simulink model "pruebaLM386"  (R2023b)
settings: Solver=VariableStepAuto  StartTime=0.0  StopTime=10.0  RelTol=1e-3
libraries: fl_lib x28, ee_lib x11, nesl_utility x3, slctrl_linear x1
settings Model: Creator=Elias  LastModifiedBy=Elias

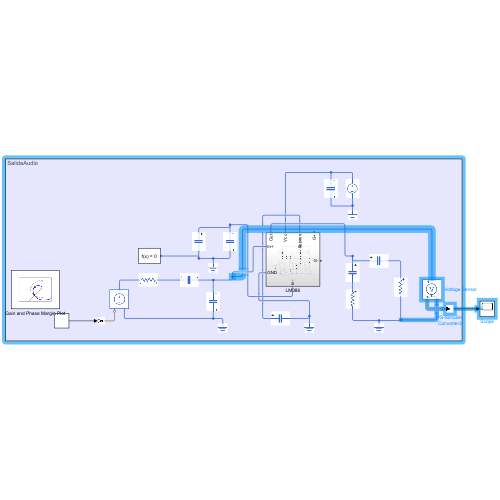
[thumbnail: Simulink's stored preview of the top-level diagram]
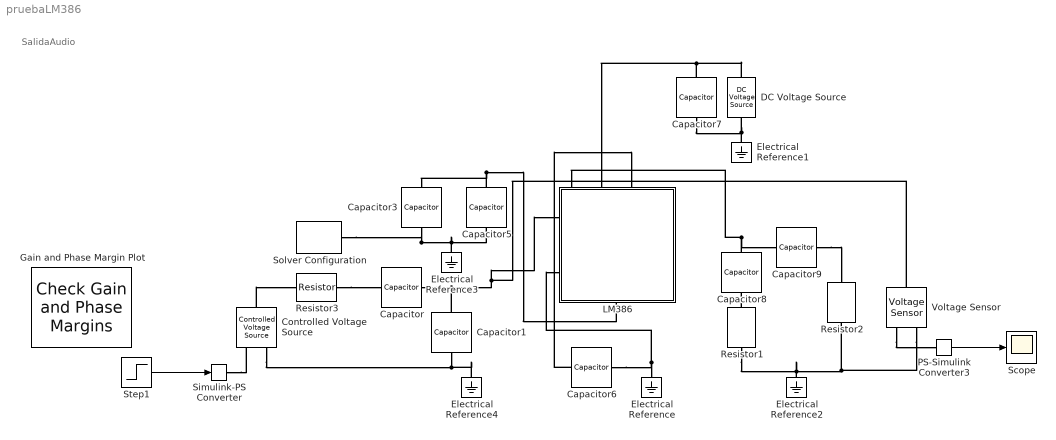
== system pruebaLM386 ==
  note: SalidaAudio
  Capacitor : fl_lib/Electrical/Electrical Elements/Capacitor  c=470e-9 F  r=0 Ohm  g=0 1/Ohm  i_specify=off  i_priority=None  i=0 A  i_nominal_specify=off  i_nominal_unit=A  i_nominal_value=1  v_specify=off  v_priority=None  v=0 V  v_nominal_specify=off  v_nominal_unit=V  v_nominal_value=1  vc_specify=off  vc_priority=High  vc=0 V  vc_nominal_specify=off  vc_nominal_unit=V  vc_nominal_value=1
  Capacitor1 : fl_lib/Electrical/Electrical Elements/Capacitor  c=1e-9 F  r=0 Ohm  g=0 1/Ohm  i_specify=off  i_priority=None  i=0 A  i_nominal_specify=off  i_nominal_unit=A  i_nominal_value=1  v_specify=off  v_priority=None  v=0 V  v_nominal_specify=off  v_nominal_unit=V  v_nominal_value=1  vc_specify=off  vc_priority=High  vc=0 V  vc_nominal_specify=off  vc_nominal_unit=V  vc_nominal_value=1
  Capacitor3 : fl_lib/Electrical/Electrical Elements/Capacitor  c=470e-9 F  r=0 Ohm  g=0 1/Ohm  i_specify=off  i_priority=None  i=0 A  i_nominal_specify=off  i_nominal_unit=A  i_nominal_value=1  v_specify=off  v_priority=None  v=0 V  v_nominal_specify=off  v_nominal_unit=V  v_nominal_value=1  vc_specify=off  vc_priority=High  vc=0 V  vc_nominal_specify=off  vc_nominal_unit=V  vc_nominal_value=1
  Capacitor5 : fl_lib/Electrical/Electrical Elements/Capacitor  c=1e-9 F  r=0 Ohm  g=0 1/Ohm  i_specify=off  i_priority=None  i=0 A  i_nominal_specify=off  i_nominal_unit=A  i_nominal_value=1  v_specify=off  v_priority=None  v=0 V  v_nominal_specify=off  v_nominal_unit=V  v_nominal_value=1  vc_specify=off  vc_priority=High  vc=0 V  vc_nominal_specify=off  vc_nominal_unit=V  vc_nominal_value=1
  Capacitor6 : fl_lib/Electrical/Electrical Elements/Capacitor  c=100e-6 F  r=0 Ohm  g=0 1/Ohm  i_specify=off  i_priority=None  i=0 A  i_nominal_specify=off  i_nominal_unit=A  i_nominal_value=1  v_specify=off  v_priority=None  v=0 V  v_nominal_specify=off  v_nominal_unit=V  v_nominal_value=1  vc_specify=off  vc_priority=High  vc=0 V  vc_nominal_specify=off  vc_nominal_unit=V  vc_nominal_value=1
  Capacitor7 : fl_lib/Electrical/Electrical Elements/Capacitor  c=100e-6 F  r=0 Ohm  g=0 1/Ohm  i_specify=off  i_priority=None  i=0 A  i_nominal_specify=off  i_nominal_unit=A  i_nominal_value=1  v_specify=off  v_priority=None  v=0 V  v_nominal_specify=off  v_nominal_unit=V  v_nominal_value=1  vc_specify=off  vc_priority=High  vc=0 V  vc_nominal_specify=off  vc_nominal_unit=V  vc_nominal_value=1
  Capacitor8 : fl_lib/Electrical/Electrical Elements/Capacitor  c=47e-6 F  r=0 Ohm  g=0 1/Ohm  i_specify=off  i_priority=None  i=0 A  i_nominal_specify=off  i_nominal_unit=A  i_nominal_value=1  v_specify=off  v_priority=None  v=0 V  v_nominal_specify=off  v_nominal_unit=V  v_nominal_value=1  vc_specify=off  vc_priority=High  vc=0 V  vc_nominal_specify=off  vc_nominal_unit=V  vc_nominal_value=1
  Capacitor9 : fl_lib/Electrical/Electrical Elements/Capacitor  c=3.3e-3 F  r=0 Ohm  g=0 1/Ohm  i_specify=off  i_priority=None  i=0 A  i_nominal_specify=off  i_nominal_unit=A  i_nominal_value=1  v_specify=off  v_priority=None  v=0 V  v_nominal_specify=off  v_nominal_unit=V  v_nominal_value=1  vc_specify=off  vc_priority=High  vc=0 V  vc_nominal_specify=off  vc_nominal_unit=V  vc_nominal_value=1
  Controlled Voltage Source : fl_lib/Electrical/Electrical Sources/Controlled Voltage Source
  DC Voltage Source : fl_lib/Electrical/Electrical Sources/DC Voltage Source  v0=5 V
  Electrical Reference{,1..4} (5 alike) : fl_lib/Electrical/Electrical Elements/Electrical Reference
  Gain and Phase Margin Plot : slctrl_linear/Check Gain and Phase Margins  InstantiateOnLoad=on  SaveOperatingPoints=off  LinearizationIOs={'/Step1', 1, 'in', 'off', '';'/PS-Simulink Converter3', 1, 'out', 'on', ''}  LinearizeAt=SnapshotTimes  SnapshotTimes=[0]  TriggerType=rising  SampleTime=auto  RateConversionMethod=zoh  PreWarpFreq=10  UseExactDelayModel=off  UseFullBlockNameLabels=off  UseBusSignalLabels=off  enabled=on  stopWhenAssertionFail=off  export=off  ViewDlgPos=[1 49 1536 740.8]  LaunchViewOnOpen=off  OpenViewOnLoad=on  FrequencyUnits=rad/s  MagnitudeUnits=dB  PhaseUnits=deg  TimeUnits=seconds  EnableMargins=off  GainMargin=[]  PhaseMargin=[]  PlotType=bode  FeedbackSign=-1
      settings: LibrarySourceBlock=slctrlblks/Linear Analysis Plots/Gain and Phase Margin Plot  SaveToWorkspace=off  SaveName=sys
  LM386 : Subsystem
      settings: PortSchema="{\"entries\":[{\"content\":{\"sides\":[{\"content\":{\"connectorIds\":[\"LConn1\",\"LConn2\"]},\"type\":\"ConnectorPlacement.EquallySpacedRectSide\",\"uuid\":\"2337400e-b5e6-493f-9361-1980809f2d02\"},{\"content\":{\"connectorIds\":[\"RConn1\"],\"side\":\"RIGHT\"},\"type\":\"ConnectorPlacement.EquallySpacedRectSide\",\"uuid\":\"8454aa5c-1d69-40e4-a810-e77be7f85d5b\"},{\"content\":{\"connectorIds\":[\"LConn3\",\"LConn4\",\"LConn5\",\"LConn6\"],\"side\":\"TOP\"},\"type\":\"ConnectorPlacement.EquallySpacedRectSide\",\"uuid\":\"a2e8fa12-598a-43b9-9543-b1b71967ef13\"},{\"content\":{\"connectorIds\":[\"RConn2\"],\"side\":\"BOTTOM\"},\"type\":\"ConnectorPlacement.EquallySpacedRectSide\",\"uuid\":\"694fd00f-bc4d-4e22-a44d-beff6c6d18ee\"}]},\"type\":\"ConnectorPlacement.EquallySpacedConnector\",\"uuid\":\"d8918919-7b49-430f-8ddf-b4266ff1b5a4\"}],\"packageUris\":[\"http://schema.mathworks.com/mf0/Connector/R2020b\"],\"version\":\"1.0\"}"
  PS-Simulink Converter3 : nesl_utility/PS-Simulink Converter  PhysicalDomain=network_engine_domain  SubClassName=ps_output  LeftPortType=input  RightPortType=output  PseudoPeriodic=off  Frequencies=[]  VectorFormat=inherit  Unit=inherit  AffineConversion=off
  Resistor1 : fl_lib/Electrical/Electrical Elements/Resistor  R=10 Ohm  i_specify=off  i_priority=None  i=0 A  i_nominal_specify=off  i_nominal_unit=A  i_nominal_value=1  v_specify=off  v_priority=None  v=0 V  v_nominal_specify=off  v_nominal_unit=V  v_nominal_value=1
  Resistor2 : fl_lib/Electrical/Electrical Elements/Resistor  R=8 Ohm  i_specify=off  i_priority=None  i=0 A  i_nominal_specify=off  i_nominal_unit=A  i_nominal_value=1  v_specify=off  v_priority=None  v=0 V  v_nominal_specify=off  v_nominal_unit=V  v_nominal_value=1
  Resistor3 : fl_lib/Electrical/Electrical Elements/Resistor  R=47 Ohm  i_specify=off  i_priority=None  i=0 A  i_nominal_specify=off  i_nominal_unit=A  i_nominal_value=1  v_specify=off  v_priority=None  v=0 V  v_nominal_specify=off  v_nominal_unit=V  v_nominal_value=1
  Scope : Scope
  Simulink-PS Converter : nesl_utility/Simulink-PS Converter  PhysicalDomain=network_engine_domain  SubClassName=ps_input  LeftPortType=input  RightPortType=output  PseudoPeriodic=off  Frequencies=[]  NoiseDistribution=none  NoiseParameters=[]  Unit=1  AffineConversion=on  FilteringAndDerivatives=filter  SimscapeFilterOrder=1  InputFilterTimeConstant=0.001  UdotUserProvided=0
  Solver Configuration : nesl_utility/Solver Configuration  PhysicalDomain=network_engine_domain  SubClassName=solver  LeftPortType=input  RightPortType=generic  Tones=[]  Harmonics=[]  SimulateNoise=off  Profile=off  UseLocalSampling=off  EnableSwitchedLinearOptims=on  FrequencyDomain=off  UseCCode=off  RelTol=0.001  AbsTol=0.001  MinStep=1e-09  ToWorkspace=off  RevertToSquareIcSolve=off  NumHomotopyIterations=100  PhasorMode=off  PhasorModeNumHarmonics=1  ConsistencySolver=NEWTON_XTOL_AFTER_FTOL  IndexReductionMethod=DerivativeReplacement  DoDC=off  ResidualTolerance=1e-09  ConsistencyTolSource=GLOBAL  ConsistencyAbsTol=0.001  ConsistencyRelTol=0.001  ConsistencyTolFactor=0.001  UseLocalSolver=off  LocalSolverChoice=NE_BACKWARD_EULER_ADVANCER  ResolveIndetEquations=on  FunctionEvalNumThread=1  LocalSolverSampleTime=0.001  DoFixedCost=off  MaxNonlinIter=3  MaxModeIter=2  ComputeImpulses=off  ImpulseIterations=2  LinearAlgebra=auto  LinearAlgebraNumThread=0  EquationFormulation=NE_TIME_EF  DelaysMemoryBudget=1024  AutomaticFiltering=on  FilteringTimeConstant=0.001  PartitionStorageMethod=AS_NEEDED  PartitionMemoryBudget=1024  PartitionMethod=ROBUST  MultibodyUseLocalSolver=off  MultibodyLocalSolverChoice=ODE1  MultibodyLocalSolverSampleTime=0.001
  Step1 : Step  SampleTime=0
  Voltage Sensor : fl_lib/Electrical/Electrical Sensors/Voltage Sensor
  wires:
  Step1/1 -> Simulink-PS Converter/1
  PS-Simulink Converter3/1 -> Scope/1
  connections:
  Simulink-PS Converter/RConn1 -- Controlled Voltage Source/RConn1
  DC Voltage Source/LConn1 -- LM386/LConn4 -- Capacitor7/LConn1
  Capacitor/RConn1 -- Capacitor1/LConn1 -- Voltage Sensor/LConn1 -- LM386/LConn1
  Capacitor6/RConn1 -- LM386/LConn2 -- Electrical Reference/LConn1
  Capacitor5/LConn1 -- Capacitor3/LConn1 -- LM386/RConn2
  Voltage Sensor/RConn1 -- PS-Simulink Converter3/LConn1
  Electrical Reference1/LConn1 -- Capacitor7/RConn1 -- DC Voltage Source/RConn1
  Capacitor6/LConn1 -- LM386/LConn5
  Capacitor8/LConn1 -- Capacitor9/LConn1 -- LM386/LConn3
  Capacitor1/RConn1 -- Electrical Reference4/LConn1 -- Controlled Voltage Source/RConn2
  Capacitor3/RConn1 -- Solver Configuration/RConn1 -- Electrical Reference3/LConn1 -- Capacitor5/RConn1
  Capacitor9/RConn1 -- Resistor2/LConn1
  Resistor1/LConn1 -- Capacitor8/RConn1
  Resistor1/RConn1 -- Electrical Reference2/LConn1 -- Voltage Sensor/RConn2 -- Resistor2/RConn1
  Controlled Voltage Source/LConn1 -- Resistor3/RConn1
  Resistor3/LConn1 -- Capacitor/LConn1

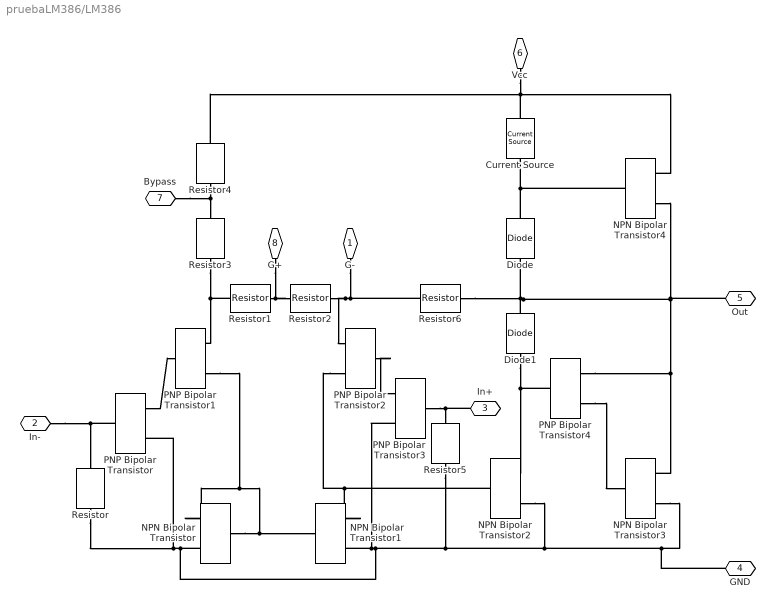
== system pruebaLM386/LM386 ==
  Current Source : ee_lib/Sources/Current Source  dc_current=5e-3 A  ac_current=0 A  ac_shift=0 rad  ac_frequency=0 Hz  noise_mode=ee.enum.sources.noise.Disabled  PSD=0 A^2/Hz  sample_time=1e-3 s  repeatability=ee.enum.sources.repeatability.NotRepeatable  user_seed=0  auto_seed=3890346746  i_specify=off  i_priority=None  i=0 A  i_nominal_specify=off  i_nominal_unit=A  i_nominal_value=1  v_specify=off  v_priority=None  v=0 V  v_nominal_specify=off  v_nominal_unit=V  v_nominal_value=1
  Diode : fl_lib/Electrical/Electrical Elements/Diode  Vf=0.6 V  Ron=0.3 Ohm  Goff=1e-8 1/Ohm  i_specify=off  i_priority=None  i=0 A  i_nominal_specify=off  i_nominal_unit=A  i_nominal_value=1  v_specify=off  v_priority=None  v=0 V  v_nominal_specify=off  v_nominal_unit=V  v_nominal_value=1
  Diode1 : fl_lib/Electrical/Electrical Elements/Diode  Vf=0.6 V  Ron=0.3 Ohm  Goff=1e-8 1/Ohm  i_specify=off  i_priority=None  i=0 A  i_nominal_specify=off  i_nominal_unit=A  i_nominal_value=1  v_specify=off  v_priority=None  v=0 V  v_nominal_specify=off  v_nominal_unit=V  v_nominal_value=1
  NPN Bipolar Transistor{,1..4} (5 alike) : ee_lib/Semiconductors & Converters/NPN Bipolar Transistor  parameterization=1  BF=100  IS=1e-14 A  VAF=200 V  hfe=100  hoe=50e-6 1/Ohm  Ic_h=1 mA  Vce_h=5 V  V1=0.55 V  I1=0.5 mA  BR=1  Tmeas=25 degC  RC=0.01 Ohm  RE=1e-4 Ohm  RB=1 Ohm  C_BC=5 pF  C_BE=5 pF  TF=0 us  TR=0 us  prmDatasheet=1  prmEquCoeff=1  hfe_T2=125  XTB=0  V1_T2=0.45 V  I1_T2=0.5 mA  Tmeas2=125 degC  EG=1.11 eV  XTI=3  TdeviceDatasheet=25 degC  TdeviceEquCoeff=25 degC  ec=1  ib_specify=off  ib_priority=None  ib=0 A  ib_nominal_specify=off  ib_nominal_unit=A  ib_nominal_value=1  ic_specify=off  ic_priority=None  ic=0 A  ic_nominal_specify=off  ic_nominal_unit=A  ic_nominal_value=1  vce_specify=off  vce_priority=None  vce=0 V  vce_nominal_specify=off  vce_nominal_unit=V  vce_nominal_value=1  vbe_specify=off  vbe_priority=None  vbe=0 V  vbe_nominal_specify=off  vbe_nominal_unit=V  vbe_nominal_value=1  v_capacitor_bc_specify=off  v_capacitor_bc_priority=High  v_capacitor_bc=0 V  v_capacitor_bc_nominal_specify=off  v_capacitor_bc_nominal_unit=V  v_capacitor_bc_nominal_value=1  v_capacitor_be_specify=off  v_capacitor_be_priority=High  v_capacitor_be=0 V  v_capacitor_be_nominal_specify=off  v_capacitor_be_nominal_unit=V  v_capacitor_be_nominal_value=1  thermal_network_parameterization=ee.enum.thermalNetworkTopology.junctionCase  Rth=[0, 10] K/W  Rth_Cauer=[1, 3, 10] K/W  Rth_Foster=[4, 6] K/W  thermal_mass_parameterization=ee.enum.thermalNetwork.timeconstant  thermal_mass=[0, 1] J/K  thermal_mass_Cauer=[.1, .3, 1] J/K  thermal_mass_Foster=[1.5, 3] J/K  thermal_time_constant=[0, 10] s  thermal_time_constant_Cauer=[1, 3, 10] s  thermal_time_constant_Foster=[6, 18] s  thermal_mass_initial_temperatures=[25, 25] degC  thermal_mass_initial_temperatures_Cauer=[25, 25, 25] degC  Tvec_initial_Foster=[25, 25, 25, 25] degC
  PNP Bipolar Transistor{,1..4} (5 alike) : ee_lib/Semiconductors & Converters/PNP Bipolar Transistor  parameterization=1  BF=100  IS=1e-14 A  VAF=200 V  hfe=100  hoe=50e-6 1/Ohm  Ic_h=-1 mA  Vce_h=-5 V  V1=-0.55 V  I1=-0.5 mA  BR=1  Tmeas=25 degC  RC=0.01 Ohm  RE=1e-4 Ohm  RB=1 Ohm  C_BC=5 pF  C_BE=5 pF  TF=0 us  TR=0 us  prmDatasheet=1  prmEquCoeff=1  hfe_T2=125  XTB=0  V1_T2=-0.45 V  I1_T2=-0.5 mA  Tmeas2=125 degC  EG=1.11 eV  XTI=3  TdeviceDatasheet=25 degC  TdeviceEquCoeff=25 degC  ec=1  ib_specify=off  ib_priority=None  ib=0 A  ib_nominal_specify=off  ib_nominal_unit=A  ib_nominal_value=1  ic_specify=off  ic_priority=None  ic=0 A  ic_nominal_specify=off  ic_nominal_unit=A  ic_nominal_value=1  vce_specify=off  vce_priority=None  vce=0 V  vce_nominal_specify=off  vce_nominal_unit=V  vce_nominal_value=1  vbe_specify=off  vbe_priority=None  vbe=0 V  vbe_nominal_specify=off  vbe_nominal_unit=V  vbe_nominal_value=1  v_capacitor_bc_specify=off  v_capacitor_bc_priority=High  v_capacitor_bc=0 V  v_capacitor_bc_nominal_specify=off  v_capacitor_bc_nominal_unit=V  v_capacitor_bc_nominal_value=1  v_capacitor_be_specify=off  v_capacitor_be_priority=High  v_capacitor_be=0 V  v_capacitor_be_nominal_specify=off  v_capacitor_be_nominal_unit=V  v_capacitor_be_nominal_value=1  thermal_network_parameterization=ee.enum.thermalNetworkTopology.junctionCase  Rth=[0, 10] K/W  Rth_Cauer=[1, 3, 10] K/W  Rth_Foster=[4, 6] K/W  thermal_mass_parameterization=ee.enum.thermalNetwork.timeconstant  thermal_mass=[0, 1] J/K  thermal_mass_Cauer=[.1, .3, 1] J/K  thermal_mass_Foster=[1.5, 3] J/K  thermal_time_constant=[0, 10] s  thermal_time_constant_Cauer=[1, 3, 10] s  thermal_time_constant_Foster=[6, 18] s  thermal_mass_initial_temperatures=[25, 25] degC  thermal_mass_initial_temperatures_Cauer=[25, 25, 25] degC  Tvec_initial_Foster=[25, 25, 25, 25] degC
      settings: InternalSimscapePortConfiguration="{\"Bottom\":[],\"Left\":[{\"id\":\"B\",\"label\":\"\",\"type\":\"foundation.electrical.electrical\"}],\"Right\":[{\"id\":\"n\",\"label\":\"\",\"type\":\"foundation.electrical.electrical\"},{\"id\":\"p\",\"label\":\"\",\"type\":\"foundation.electrical.electrical\"}],\"Top\":[]}"
  Resistor : fl_lib/Electrical/Electrical Elements/Resistor  R=50e3 Ohm  i_specify=off  i_priority=None  i=0 A  i_nominal_specify=off  i_nominal_unit=A  i_nominal_value=1  v_specify=off  v_priority=None  v=0 V  v_nominal_specify=off  v_nominal_unit=V  v_nominal_value=1
  Resistor1 : fl_lib/Electrical/Electrical Elements/Resistor  R=150 Ohm  i_specify=off  i_priority=None  i=0 A  i_nominal_specify=off  i_nominal_unit=A  i_nominal_value=1  v_specify=off  v_priority=None  v=0 V  v_nominal_specify=off  v_nominal_unit=V  v_nominal_value=1
  Resistor2 : fl_lib/Electrical/Electrical Elements/Resistor  R=1.35e3 Ohm  i_specify=off  i_priority=None  i=0 A  i_nominal_specify=off  i_nominal_unit=A  i_nominal_value=1  v_specify=off  v_priority=None  v=0 V  v_nominal_specify=off  v_nominal_unit=V  v_nominal_value=1
  Resistor3 : fl_lib/Electrical/Electrical Elements/Resistor  R=15e3 Ohm  i_specify=off  i_priority=None  i=0 A  i_nominal_specify=off  i_nominal_unit=A  i_nominal_value=1  v_specify=off  v_priority=None  v=0 V  v_nominal_specify=off  v_nominal_unit=V  v_nominal_value=1
  Resistor4 : fl_lib/Electrical/Electrical Elements/Resistor  R=15e3 Ohm  i_specify=off  i_priority=None  i=0 A  i_nominal_specify=off  i_nominal_unit=A  i_nominal_value=1  v_specify=off  v_priority=None  v=0 V  v_nominal_specify=off  v_nominal_unit=V  v_nominal_value=1
  Resistor5 : fl_lib/Electrical/Electrical Elements/Resistor  R=50e3 Ohm  i_specify=off  i_priority=None  i=0 A  i_nominal_specify=off  i_nominal_unit=A  i_nominal_value=1  v_specify=off  v_priority=None  v=0 V  v_nominal_specify=off  v_nominal_unit=V  v_nominal_value=1
  Resistor6 : fl_lib/Electrical/Electrical Elements/Resistor  R=1 Ohm  i_specify=off  i_priority=None  i=0 A  i_nominal_specify=off  i_nominal_unit=A  i_nominal_value=1  v_specify=off  v_priority=None  v=0 V  v_nominal_specify=off  v_nominal_unit=V  v_nominal_value=1
  G- : PMIOPort  Side=Right
  In- : PMIOPort  Port=2  Side=Right
  In+ : PMIOPort  Port=3  Side=Left
  GND : PMIOPort  Port=4  Side=Left
  Out : PMIOPort  Port=5  Side=Left
  Vcc : PMIOPort  Port=6  Side=Left
  Bypass : PMIOPort  Port=7  Side=Left
  G+ : PMIOPort  Port=8  Side=Left
  connections:
  NPN Bipolar Transistor/RConn1 -- NPN Bipolar Transistor/LConn1 -- NPN Bipolar Transistor1/LConn1 -- PNP Bipolar Transistor1/RConn2
  Current Source/LConn1 -- Diode/LConn1 -- NPN Bipolar Transistor4/LConn1
  Resistor4/RConn1 -- Bypass/RConn1 -- Resistor3/LConn1
  Resistor3/RConn1 -- Resistor1/LConn1 -- PNP Bipolar Transistor1/RConn1
  PNP Bipolar Transistor3/LConn1 -- In+/RConn1 -- Resistor5/LConn1
  Resistor1/RConn1 -- G+/RConn1 -- Resistor2/LConn1
  PNP Bipolar Transistor4/RConn2 -- NPN Bipolar Transistor3/LConn1
  PNP Bipolar Transistor3/RConn2 -- NPN Bipolar Transistor1/RConn2 -- NPN Bipolar Transistor/RConn2 -- Resistor/RConn1 -- PNP Bipolar Transistor/RConn2 -- GND/RConn1 -- NPN Bipolar Transistor3/RConn2 -- NPN Bipolar Transistor2/RConn2 -- Resistor5/RConn1
  PNP Bipolar Transistor4/LConn1 -- Diode1/RConn1 -- NPN Bipolar Transistor2/RConn1
  Diode1/LConn1 -- Diode/RConn1 -- Out/RConn1 -- NPN Bipolar Transistor4/RConn2 -- PNP Bipolar Transistor4/RConn1 -- NPN Bipolar Transistor3/RConn1 -- Resistor6/RConn1
  Resistor4/LConn1 -- Vcc/RConn1 -- Current Source/RConn1 -- NPN Bipolar Transistor4/RConn1
  PNP Bipolar Transistor2/RConn2 -- NPN Bipolar Transistor1/RConn1 -- NPN Bipolar Transistor2/LConn1
  PNP Bipolar Transistor/LConn1 -- In-/RConn1 -- Resistor/LConn1
  PNP Bipolar Transistor/RConn1 -- PNP Bipolar Transistor1/LConn1
  Resistor6/LConn1 -- G-/RConn1 -- Resistor2/RConn1 -- PNP Bipolar Transistor2/RConn1
  PNP Bipolar Transistor2/LConn1 -- PNP Bipolar Transistor3/RConn1
